simulink model "FreqMeter"  (R2026a)
settings: Solver=FixedStepDiscrete  StopTime=inf  FixedStep=Ts
model workspace (MATLAB code in the model file):
  | % Defaults for standalone use, from HPP_parameters. In HPP the Model
  | % block passes the instance's parameters as the argument "m".
  | pDefault = HPP_parameters();
  | Ts = pDefault.sim.Ts;      % [s] simulation step
  | m = pDefault.pll.hppc;
  | clear pDefault
Description:
  | Frequency meter: PLL, frequency averaged over Navg steps (m.on = 0: f_sys), RoCoF over Nroc steps. Argument m: see params/pllParameters.m.
settings Model: ParameterArgumentNames=m  Creator=kjaer  LastModifiedBy=kjaer

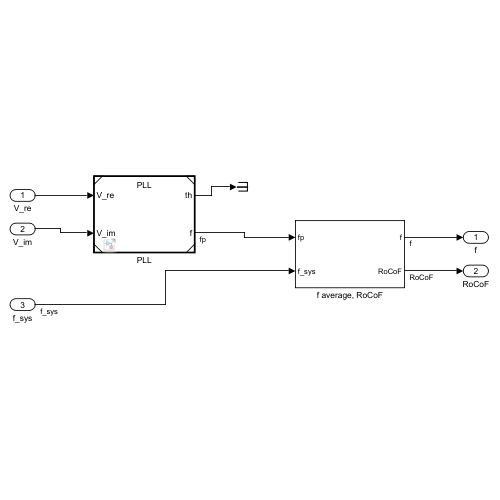
[thumbnail: Simulink's stored preview of the top-level diagram]
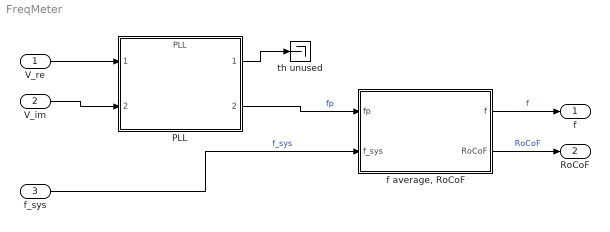
== system FreqMeter ==
  V_re : Inport
  V_im : Inport  Port=2
  f_sys : Inport  Port=3
  PLL : ModelReference  ModelNameDialog=PLL  ParameterArgumentNames=pll  ParameterArgumentValues=m  UsingDefaultArgumentValue=0  SimulationMode=Normal  ModelReferenceVersion=1.1
  "f average, RoCoF" : Subsystem  Description=f = moving average of the PLL frequency over Navg steps (on = 0: f_sys); RoCoF over Nroc steps
  th unused : Terminator
  f : Outport
  RoCoF : Outport  Port=2
  wires:
  V_re/1 -> PLL/1
  V_im/1 -> PLL/2
  PLL/1 -> th unused/1
  PLL/2 -> "f average, RoCoF"/1(fp)  "fp"
  f_sys/1 -> "f average, RoCoF"/2(f_sys)  "f_sys"
  "f average, RoCoF"/1(f) -> f/1  "f"
  "f average, RoCoF"/2(RoCoF) -> RoCoF/1  "RoCoF"

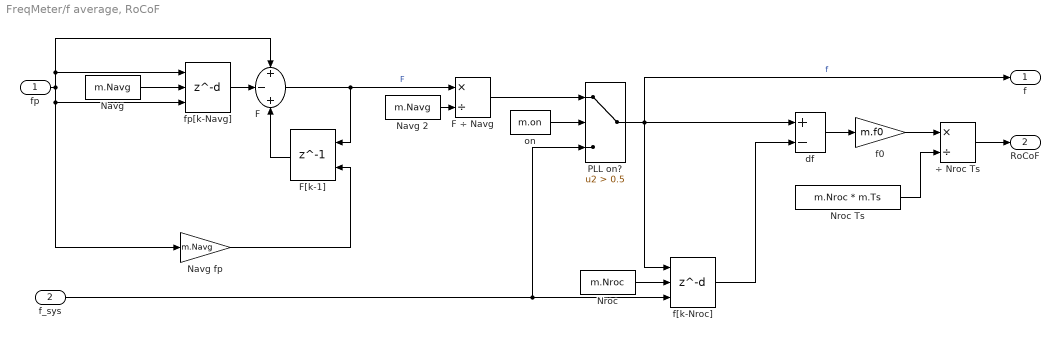
== system FreqMeter/f average, RoCoF ==
  fp : Inport
  f_sys : Inport  Port=2
  F : Sum  Inputs=+-+
  F ÷ Navg : Product  Inputs=*/
  F[k-1] : Delay  DelayLength=1  InitialConditionSource=Input port
      settings: InputPortMap=u0,p4
  Navg : Constant  Value=m.Navg
  Navg 2 : Constant  Value=m.Navg
  Navg fp : Gain  Gain=m.Navg
  Nroc : Constant  Value=m.Nroc
  Nroc Ts : Constant  Value=m.Nroc * m.Ts
  PLL on? : Switch  Criteria=u2 > Threshold  Threshold=0.5  SaturateOnIntegerOverflow=off  InputSameDT=off
  df : Sum  Inputs=+-
  f0 : Gain  Gain=m.f0
  f[k-Nroc] : Delay  DelayLengthSource=Input port  DelayLengthUpperLimit=1000  InitialConditionSource=Input port
      settings: InputPortMap=u0,p1,p4
  fp[k-Navg] : Delay  DelayLengthSource=Input port  DelayLengthUpperLimit=50  InitialConditionSource=Input port
      settings: InputPortMap=u0,p1,p4
  on : Constant  Value=m.on
  ÷ Nroc Ts : Product  Inputs=*/
  f : Outport
  RoCoF : Outport  Port=2
  wires:
  ÷ Nroc Ts/1 -> RoCoF/1
  Nroc Ts/1 -> ÷ Nroc Ts/2
  f0/1 -> ÷ Nroc Ts/1
  df/1 -> f0/1
  f[k-Nroc]/1 -> df/2
  Nroc/1 -> f[k-Nroc]/2
  PLL on?/1 -> f[k-Nroc]/1, df/1, f/1  "f"
  f_sys/1 -> f[k-Nroc]/3, PLL on?/3
  on/1 -> PLL on?/2
  F ÷ Navg/1 -> PLL on?/1
  Navg 2/1 -> F ÷ Navg/2
  Navg fp/1 -> F[k-1]/2
  F[k-1]/1 -> F/3
  F/1 -> F ÷ Navg/1, F[k-1]/1  "F"
  fp[k-Navg]/1 -> F/2
  Navg/1 -> fp[k-Navg]/2
  fp/1 -> fp[k-Navg]/3, Navg fp/1, F/1, fp[k-Navg]/1
